simulink model "Single_Phase_Half_3_Level_FCNPC_Rectifier"  (R2023b)
settings: Solver=VariableStepAuto  StartTime=0.0  StopTime=0.5  RelTol=1e-3
libraries: spsVoltageMeasurementLib x5, spsSeriesRLCBranchLib x4, spsIGBTDiodeLib x4, spsMosfetLib x2, spsACVoltageSourceLib x1, spsCurrentMeasurementLib x1, spsMeanLib x1, slpidlib x1, powerlib_extras x1, spsRMSLib x1, spsTHDLib x1, spspowerguiLib x1
settings Model: SimulationMode=accelerator  Creator=abc6820292  LastModifiedBy=45276
settings DataIOCC: ReturnWorkspaceOutputs=off
settings DebuggingCC: UnconnectedInputMsg=warning  UnconnectedOutputMsg=warning  UnconnectedLineMsg=warning
settings ModelReferenceCC: EnableRefExpFcnMdlSchedulingChecks=on
settings RTWCC: DLArmComputeVersion=19.05

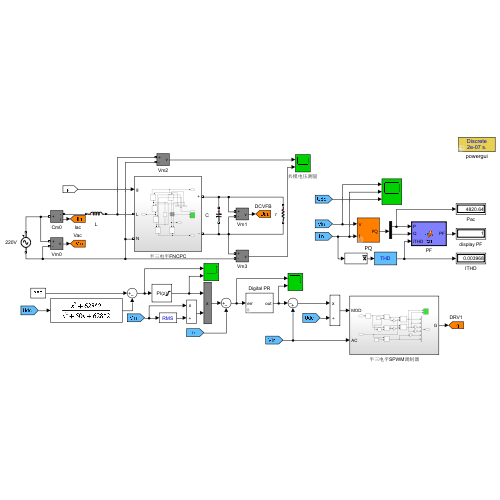
[thumbnail: Simulink's stored preview of the top-level diagram]
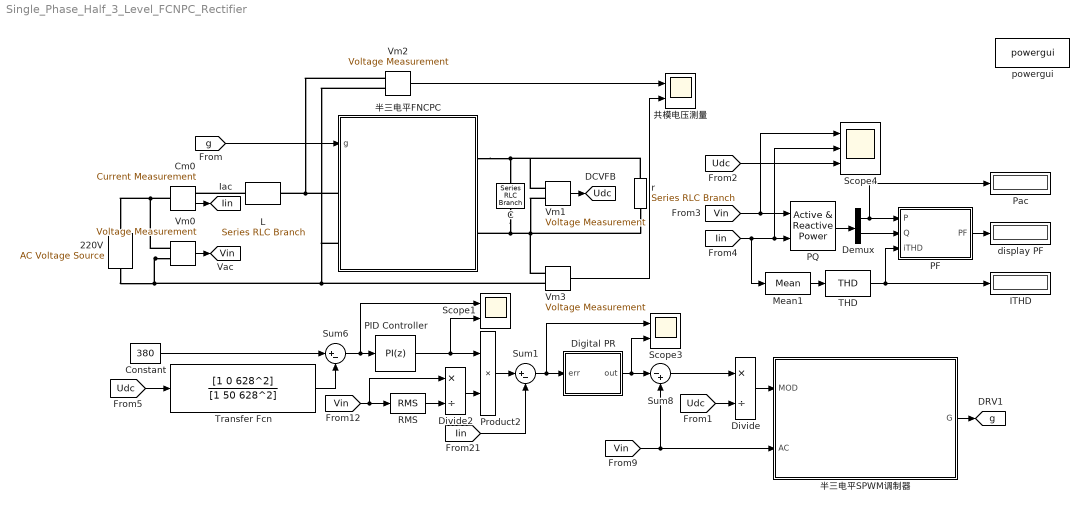
== system Single_Phase_Half_3_Level_FCNPC_Rectifier ==
  220V : spsACVoltageSourceLib/AC Voltage Source  Amplitude=220*1.414  Phase=0  Frequency=50  SampleTime=0  Measurements=None  BusType=swing  Pref=10e3  Qref=0  Qmin=-inf  Qmax=+inf
  C : spsSeriesRLCBranchLib/Series RLC Branch  LConnTagsString=__new0  RConnTagsString=__new0  BranchType=C  Resistance=0.01  Inductance=7e-4  SetiL0=off  InitialCurrent=0  Capacitance=2e-3  Setx0=on  InitialVoltage=360  Measurements=None
  Cm0 : spsCurrentMeasurementLib/Current Measurement  PhasorSimulation=off  OutputType=Complex  PSBequivalent=0
  Constant : Constant  Value=380
  Demux : Demux  Outputs=2
  Digital PR : Subsystem  mask{Kp=4, Kr=100, Wc=5, Ts=1/40000, Upper=400, Lower=-400}
      mask DialogControl ParameterGroupVar Prompt: 参数
  Divide : Product  Inputs=*/
  Divide2 : Product  Inputs=*/
  ITHD : Display
  L : spsSeriesRLCBranchLib/Series RLC Branch  LConnTagsString=__new0  RConnTagsString=__new0  BranchType=L  Resistance=0.05  Inductance=6e-4  SetiL0=off  InitialCurrent=0  Capacitance=1e-3  Setx0=off  InitialVoltage=0  Measurements=None
  Mean1 : spsMeanLib/Mean  Freq=10000  Vinit=0  Ts=0
  PF : MATLAB Function  TreatAsAtomicUnit=on
  PID Controller : slpidlib/PID Controller  Controller=PI  Form=Parallel  TimeDomain=Discrete-time  UseExternalTs=off  SampleTime=1/40000  IntegratorMethod=Forward Euler  FilterMethod=Forward Euler  ControllerParametersSource=internal  P=0.2  I=10  UseKiTs=off  D=0.005  N=100  UseFilter=on  TunerSelectOption=Transfer Function Based (PID Tuner App)  InitialConditionSource=internal  InitialConditionForIntegrator=0  InitialConditionForFilter=0  DifferentiatorICPrevScaledInput=0  ExternalReset=none  TrackingMode=off  Kt=1  LimitOutput=on  SatLimitsSource=internal  UpperSaturationLimit=200  LowerSaturationLimit=0  LinearizeAsGain=on  AntiWindupMode=clamping  Kb=1  LimitIntegrator=off  UpperIntegratorSaturationLimit=inf  LowerIntegratorSaturationLimit=-inf  POutMin=[]  POutMax=[]  IOutMin=[]  IOutMax=[]  DOutMin=[]  DOutMax=[]  NOutMin=[]  NOutMax=[]  SumOutMin=[]  SumOutMax=[]  SaturationOutMin=[]  SaturationOutMax=[]  PParamMin=[]  PParamMax=[]  IParamMin=[]  IParamMax=[]  DParamMin=[]  DParamMax=[]  NParamMin=[]  NParamMax=[]  KbParamMin=[]  KbParamMax=[]  KtParamMin=[]  KtParamMax=[]  KbOutMin=[]  KbOutMax=[]  KtOutMin=[]  KtOutMax=[]  IntegratorOutMin=[]  IntegratorOutMax=[]  FilterOutMin=[]  FilterOutMax=[]  SumI1OutMin=[]  SumI1OutMax=[]  SumI2OutMin=[]  SumI2OutMax=[]  SumI3OutMin=[]  SumI3OutMax=[]  SumI4OutMin=[]  SumI4OutMax=[]  SumDOutMin=[]  SumDOutMax=[]  DifferentiatorOutMin=[]  DifferentiatorOutMax=[]  FilterDiffOutCoefMin=[]  FilterDiffOutCoefMax=[]  ReciprocalOutMin=[]  ReciprocalOutMax=[]  SumDenOutMin=[]  SumDenOutMax=[]  SumNumOutMin=[]  SumNumOutMax=[]  DivideOutMin=[]  DivideOutMax=[]  UdiffTsProdOutMin=[]  UdiffTsProdOutMax=[]  NTsProdOutMin=[]  NTsProdOutMax=[]  UintegralTsProdOutMin=[]  UintegralTsProdOutMax=[]  UngainTsProdOutMin=[]  UngainTsProdOutMax=[]  ClampingZeroOutDataTypeStr=Inherit: Inherit via back propagation  ClampingZeroOutMin=[]  ClampingZeroOutMax=[]  FilterDenConstantOutDataTypeStr=Inherit: Inherit via back propagation  FilterDenConstantOutMin=[]  FilterDenConstantOutMax=[]  PCopyOutDataTypeStr=Inherit: Inherit via back propagation  PCopyOutMin=[]  PCopyOutMax=[]  NCopyOutDataTypeStr=Inherit: Inherit via back propagation  NCopyOutMin=[]  NCopyOutMax=[]  IntegratorContinuousStateAttributes=''  IntegratorStateMustResolveToSignalObject=off  IntegratorRTWStateStorageClass=Auto  FilterContinuousStateAttributes=''  FilterStateMustResolveToSignalObject=off  FilterRTWStateStorageClass=Auto  ParallelPVariant=InternalParameters  IdealPVariant=Disabled  IVariant=InternalParameters  DVariant=Disabled  IntegratorVariant=Discrete  SatVariant=Enabled  AWVariant=DiscClampingParallel  PCopyVariant=Disabled  TRVariant=Disabled  FdbkBlocksVariant=Forward  IdealPFdbkVariant=Disabled  SatFdbkVariant=Disabled  DerivativeFilterVariant=Disabled  NVariant=Disabled  NCopyVariant=Disabled_SignalSpec  FilterICVariant=Disabled  IntegratorICVariant=InternalICs  ExternalResetVariant=Disabled  TRSumVariant=Passthrough  SumFdbkVariant=Disabled  SumVariant=Sum_PI  TsampFilterVariant=InternalTs  TsampNgainVariant=Passthrough  TsampIntegralVariant=Disabled_SignalSpec  ExternalSaturationOutDataTypeStr=Inherit: Same as second input
  PQ : powerlib_extras/Measurements/Active & Reactive Power  f1=50
  Pac : Display
      settings: Format=bank
  Product2 : Product  RndMeth=Zero
  RMS : spsRMSLib/RMS  TrueRMS=off  Freq=50  RMSInit=220  Ts=0
  Scope1 : Scope  NumInputPorts=2
  Scope3 : Scope  NumInputPorts=2
  Scope4 : Scope  NumInputPorts=3
  Sum1 : Sum  Inputs=|+-
  Sum6 : Sum  Inputs=|+-
  Sum8 : Sum  Inputs=|-+
  THD : spsTHDLib/THD  Freq=50  Ts=0
  Transfer Fcn : TransferFcn  Numerator=[1 0 628^2]  Denominator=[1 50 628^2]
  Vm{0..3} (4 alike) : spsVoltageMeasurementLib/Voltage Measurement  PhasorSimulation=off  OutputType=Complex  PSBequivalent=0
  display PF : Display
  powergui : spspowerguiLib/powergui  SimulationMode=Discrete  SampleTime=2e-7  frequency=60  Iterations=50  frequencyindice=0  Pbase=100e6  ErrMax=1e-4  UnitsV=kV  UnitsW=MW  buscounter=0  FunctionMessages=off  echomessages=off  EnableUseOfTLC=off  CurrentSourceSwitches=off  DisableSnubberDevices=off  DisableRonSwitches=off  DisableVfSwitches=off  DisplayEquations=off  AutomaticDiscreteSolvers=off  SolverType=Tustin/Backward Euler (TBE)  Interpol=off  ExternalGateDelay=off  methode=off  Ts=0  x0status=blocks  SPID=off  SwTol=0  HookPort=off  NonlinearTolerance=1e-4  nMaxIteration=100  ContinueOnMaxIteration=off  RestoreLinks=warning  ResistiveCurrentMeasurement=off  Frange=[0:2:500]  Ylog=off  Xlog=on  ShowGrid=off  save=off  variable=ZData  structure=QQQQQ  ZoomFFT=off  StartTime=0.5  cycles=15  DisplayStyle=1  fundamental=50  FreqAxis=off  MaxFrequency=1000  frequencyindicesteady=1  RmsSteady=1  display=off
  r : spsSeriesRLCBranchLib/Series RLC Branch  LConnTagsString=__new0  RConnTagsString=__new0  BranchType=R  Resistance=30  Inductance=1e-4  SetiL0=off  InitialCurrent=0  Capacitance=1e-3  Setx0=off  InitialVoltage=0  Measurements=None
  共模电压测量 : Scope  NumInputPorts=2
  半三电平FNCPC : Subsystem
  半三电平SPWM调制器 : Subsystem
  tag scope: Iin=global, Udc=global, Vin=global, g=global
  wires:
  Vm0/1 -> [Vin]
  Demux/2 -> PF/2(Q)
  PF/1(PF) -> display PF/1
  PQ/1 -> Demux/1
  THD/1 -> ITHD/1, PF/3(iTHD)
  [Vin] -> Scope4/1, PQ/1
  Demux/1 -> Pac/1, PF/1(P)
  Vm1/1 -> [Udc]
  半三电平SPWM调制器/1(G) -> [g]
  Divide/1 -> 半三电平SPWM调制器/1(MOD)
  [Iin] -> Sum1/2
  Sum8/1 -> Divide/1
  [Vin] -> Sum8/2, 半三电平SPWM调制器/2(AC)
  [Vin] -> RMS/1, Divide2/1
  RMS/1 -> Divide2/2
  Divide2/1 -> Product2/2
  Mean1/1 -> THD/1
  Sum1/1 -> Digital PR/1(err), Scope3/1
  Product2/1 -> Sum1/1
  Vm2/1 -> 共模电压测量/1
  Vm3/1 -> 共模电压测量/2
  Digital PR/1(out) -> Scope3/2, Sum8/1
  [g] -> 半三电平FNCPC/1(g)
  Cm0/1 -> [Iin]
  [Iin] -> Mean1/1, Scope4/2, PQ/2
  [Udc] -> Scope4/3
  [Udc] -> Divide/2
  PID Controller/1 -> Scope1/2, Product2/1
  Sum6/1 -> Scope1/1, PID Controller/1
  Transfer Fcn/1 -> Sum6/2
  [Udc] -> Transfer Fcn/1
  Constant/1 -> Sum6/1
  connections:
  半三电平FNCPC/RConn1 -- r/LConn1 -- Vm1/LConn1 -- C/LConn1
  Vm2/LConn1 -- 半三电平FNCPC/LConn1 -- L/RConn1
  Vm0/LConn2 -- Vm2/LConn2 -- 半三电平FNCPC/LConn2 -- Vm3/LConn2 -- 220V/LConn1
  L/LConn1 -- Cm0/RConn1
  Cm0/LConn1 -- 220V/RConn1 -- Vm0/LConn1
  Vm1/LConn2 -- 半三电平FNCPC/RConn2 -- C/RConn1 -- r/RConn1 -- Vm3/LConn1

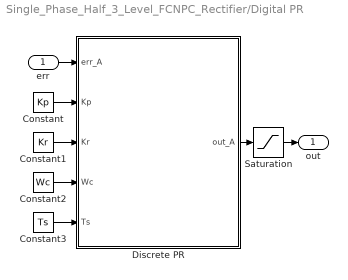
== system Single_Phase_Half_3_Level_FCNPC_Rectifier/Digital PR ==
  err : Inport
  Constant : Constant  Value=Kp
  Constant1 : Constant  Value=Kr
  Constant2 : Constant  Value=Wc
  Constant3 : Constant  Value=Ts
  Discrete PR : MATLAB Function  TreatAsAtomicUnit=on
  Saturation : Saturate  UpperLimit=Upper  LowerLimit=Lower
  out : Outport
  wires:
  Constant1/1 -> Discrete PR/3(Kr)
  Constant3/1 -> Discrete PR/5(Ts)
  Constant/1 -> Discrete PR/2(Kp)
  Constant2/1 -> Discrete PR/4(Wc)
  Discrete PR/1(out_A) -> Saturation/1
  Saturation/1 -> out/1
  err/1 -> Discrete PR/1(err_A)

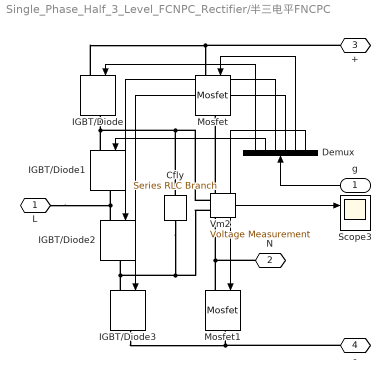
== system Single_Phase_Half_3_Level_FCNPC_Rectifier/半三电平FNCPC ==
  g : Inport
  Cfly : spsSeriesRLCBranchLib/Series RLC Branch  LConnTagsString=__new0  RConnTagsString=__new0  BranchType=C  Resistance=0.05  Inductance=6e-4  SetiL0=off  InitialCurrent=0  Capacitance=2e-5  Setx0=on  InitialVoltage=155  Measurements=None
  Demux : Demux  Outputs=6
  IGBT/Diode{,1..3} (4 alike) : spsIGBTDiodeLib/IGBT//Diode  Ron=1e-3  Rs=1e5  Cs=inf  Measurements=off
  Mosfet : spsMosfetLib/Mosfet  Ron=0.01  Lon=0  Rd=0.01  Vfd=0  IC=0  Rs=1e5  Cs=inf  Measurements=off
  Mosfet1 : spsMosfetLib/Mosfet  Ron=0.01  Lon=0  Rd=0.01  Vfd=0  IC=0  Rs=1e5  Cs=inf  Measurements=off
  Scope3 : Scope  NumInputPorts=2
  Vm2 : spsVoltageMeasurementLib/Voltage Measurement  PhasorSimulation=off  OutputType=Complex  PSBequivalent=0
  L : PMIOPort  Side=Left
  N : PMIOPort  Port=2  Side=Left
  + : PMIOPort  Port=3  Side=Right
  - : PMIOPort  Port=4  Side=Right
  wires:
  Demux/1 -> IGBT/Diode/1
  Demux/2 -> IGBT/Diode1/1
  Demux/3 -> IGBT/Diode2/1
  Demux/4 -> IGBT/Diode3/1
  Demux/5 -> Mosfet/1
  Demux/6 -> Mosfet1/1
  g/1 -> Demux/1
  Vm2/1 -> Scope3/1
  connections:
  Mosfet1/LConn1 -- Mosfet/RConn1 -- N/RConn1
  +/RConn1 -- IGBT/Diode/LConn1 -- Mosfet/LConn1
  -/RConn1 -- IGBT/Diode3/RConn1 -- Mosfet1/RConn1
  IGBT/Diode1/LConn1 -- Vm2/LConn1 -- Cfly/LConn1 -- IGBT/Diode/RConn1
  IGBT/Diode2/LConn1 -- L/RConn1 -- IGBT/Diode1/RConn1
  IGBT/Diode3/LConn1 -- Vm2/LConn2 -- Cfly/RConn1 -- IGBT/Diode2/RConn1

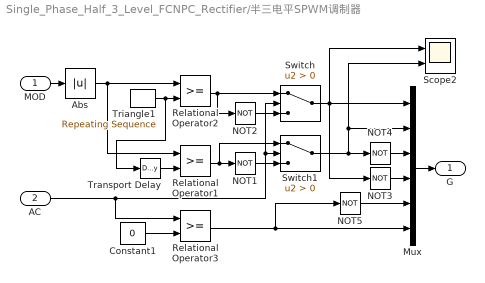
== system Single_Phase_Half_3_Level_FCNPC_Rectifier/半三电平SPWM调制器 ==
  MOD : Inport
  AC : Inport  Port=2
  Abs : Abs  SaturateOnIntegerOverflow=off
  Constant1 : Constant  Value=0
  Mux : Mux  Inputs=6
  NOT{1..5} (5 alike) : Logic  Operator=NOT  IconShape=distinctive  AllPortsSameDT=off  OutDataTypeStr=boolean
  Relational Operator1 : RelationalOperator  OutDataTypeStr=boolean  InputSameDT=off
  Relational Operator2 : RelationalOperator  OutDataTypeStr=boolean  InputSameDT=off
  Relational Operator3 : RelationalOperator  OutDataTypeStr=boolean  InputSameDT=off
  Scope2 : Scope  NumInputPorts=2
  Switch : Switch  Criteria=u2 > Threshold  SaturateOnIntegerOverflow=off  InputSameDT=off
  Switch1 : Switch  Criteria=u2 > Threshold  SaturateOnIntegerOverflow=off  InputSameDT=off
  Transport Delay : TransportDelay  DelayTime=1/20000/2
  Triangle1 : simulink/Sources/Repeating Sequence  rep_seq_t=[0 1/20000/2 1/20000]  rep_seq_y=[0 1 0]
  G : Outport
  wires:
  Mux/1 -> G/1
  MOD/1 -> Abs/1
  Abs/1 -> Relational Operator1/1, Relational Operator2/1
  Constant1/1 -> Relational Operator3/2
  NOT2/1 -> Switch/3
  Relational Operator2/1 -> NOT2/1, Switch/1
  Relational Operator1/1 -> Switch1/1, NOT1/1
  NOT1/1 -> Switch1/3
  Switch/1 -> NOT3/1, Scope2/1, Mux/1
  Switch1/1 -> Scope2/2, Mux/2, NOT4/1
  NOT5/1 -> Mux/5
  Relational Operator3/1 -> NOT5/1, Mux/6
  AC/1 -> Relational Operator3/1, Switch/2, Switch1/2
  NOT4/1 -> Mux/3
  NOT3/1 -> Mux/4
  Transport Delay/1 -> Relational Operator1/2
  Triangle1/1 -> Transport Delay/1, Relational Operator2/2

== matlab function Single_Phase_Half_3_Level_FCNPC_Rectifier/PF ==
  data: P input; PF output; Q input; iTHD input
function PF = fcn(P,Q,iTHD)
% This block supports an embeddable subset of the MATLAB language.
% See the help menu for details. 
PF=(P/sqrt(P*P+Q*Q))/(sqrt(1+iTHD*iTHD));

== matlab function Single_Phase_Half_3_Level_FCNPC_Rectifier/Digital PR/Discrete PR ==
  settings: updateMethod=DISCRETE  sampleTime=Ts
  data: err_A input; out_A output; Kp input; Kr input; Wc input; Ts input
function out_A  = fcn(err_A, Kp, Kr, Wc, Ts)

W0 = 50*2*pi;


persistent err_A1;
persistent err_A2;
persistent out_A1;
persistent out_A2;


%%对三相静态变量初始化
if isempty(err_A1)
    err_A1 = 0;
end
if isempty(err_A2)
    err_A2 = 0;
end
if isempty(out_A1)
    out_A1 = 0;
end
if isempty(out_A2)
    out_A2 = 0;
end


%%Discrete
t1 = Wc * Ts;
t2 = W0^2 * Ts^2;
t3 = t2 + 4*t1 + 4;

b0 = (Kp*t2 + 4*(Kp+Kr)*t1 + 4*Kp) / t3;
b1 = (2*Kp*t2 - 8*Kp) / t3;
b2 = (Kp*t2 + 4*Kp - 4*(Kp+Kr)*t1) / t3;
a1 = (2*t2 - 8) / t3;
a2 = (t2 - 4*t1 + 4) / t3;
%%限制输出
if b0>3000
    b0=0;
end
if b0<-3000
    b0=0;
end

%%计算输出量
out_A = b0*err_A + b1*err_A1 + b2*err_A2 - a1*out_A1 - a2*out_A2;
out_A2 = out_A1;
out_A1 = out_A;
err_A2 = err_A1;
err_A1 = err_A;
